simulink model "bms_unified"  (R2024b)
settings: Solver=FixedStepDiscrete  StartTime=0.0  StopTime=BMS_StopTime  FixedStep=1  RelTol=1e-3
InitFcn:
  | bms_setup('unified')
values from neighbouring files (symbols this model uses):
  BMS_Q : value not decoded    [bms_data.sldd]
  BMS_R = 0.001474701    [bms_data.sldd]
  NASA_Q : value not decoded    [bms_data.sldd]
  NASA_R = 0.009881778    [bms_data.sldd]
undefined symbols (not defined in the file or in its folder): BMS_FaultMode, BMS_InjectFaultsOnReplay, BMS_Seed, BMS_SOC0, BMS_SOC_Guess, BMS_Source, NASA_SOC_Guess
settings Model: DataDictionary=bms_data.sldd  Creator=sande  LastModifiedBy=sande
settings DataIOCC: SaveOutput=off
settings DebuggingCC: SignalInfNanChecking=error  AlgebraicLoopMsg=error  ArtificialAlgebraicLoopMsg=error  UnconnectedInputMsg=error  UnconnectedOutputMsg=error  UnconnectedLineMsg=error  BusObjectLabelMismatch=error  StrictBusMsg=ErrorOnBusTreatedAsVector
settings HardwareCC: ProdBitPerPointer=32  ProdBitPerSizeT=32  ProdBitPerPtrDiffT=32  ProdLargestAtomicInteger=Long  ProdLargestAtomicFloat=Double  ProdWordSize=32  ProdHWDeviceType=ARM Compatible->ARM Cortex

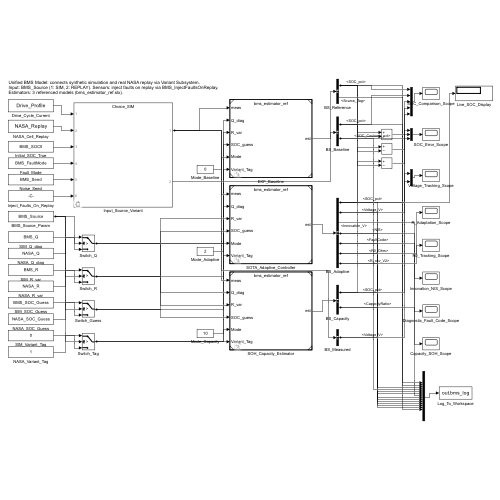
[thumbnail: Simulink's stored preview of the top-level diagram]
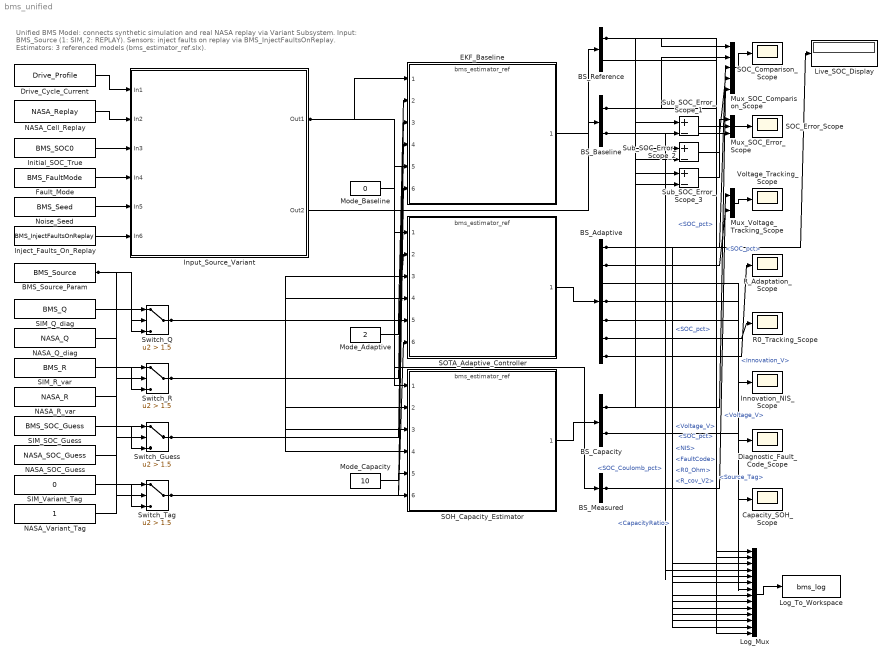
== system bms_unified ==
  note: Unified BMS Model: connects synthetic simulation and real NASA replay via Variant Subsystem.
      | Input: BMS_Source (1: SIM, 2: REPLAY). Sensors: inject faults on replay via BMS_InjectFaultsOnReplay.
      | Estimators: 3 referenced models (bms_estimator_ref.slx).
  BMS_Source_Param : Constant  Value=BMS_Source  SampleTime=-1
  BS_Adaptive : BusSelector  OutputSignals=SOC_pct,Voltage_V,Innovation_V,NIS,FaultCode,R0_Ohm,R_cov_V2
  BS_Baseline : BusSelector  OutputSignals=SOC_pct,SOC_Coulomb_pct
  BS_Capacity : BusSelector  OutputSignals=SOC_pct,CapacityRatio
  BS_Measured : BusSelector  OutputSignals=Voltage_V
  BS_Reference : BusSelector  OutputSignals=SOC_pct,Source_Tag
  Capacity_SOH_Scope : Scope
      settings: Description=Estimated capacity ratio (SOH)
  Diagnostic_Fault_Code_Scope : Scope
      settings: Description=Diagnostic bit-mask
  Drive_Cycle_Current : FromWorkspace  VariableName=Drive_Profile  SampleTime=1  Interpolate=off  OutputAfterFinalValue=Holding final value
  EKF_Baseline : ModelReference  ModelNameDialog=bms_estimator_ref  SimulationMode=Normal  ModelReferenceVersion=1.2
  Fault_Mode : Constant  Value=BMS_FaultMode  SampleTime=-1
  Initial_SOC_True : Constant  Value=BMS_SOC0  SampleTime=-1
  Inject_Faults_On_Replay : Constant  Value=BMS_InjectFaultsOnReplay  SampleTime=-1
  Innovation_NIS_Scope : Scope
      settings: Description=NIS (expect ~1)
  Input_Source_Variant : Subsystem  Variant=on
  Live_SOC_Display : Display
  Log_Mux : Mux  Inputs=14
  Log_To_Workspace : ToWorkspace  VariableName=bms_log  SampleTime=-1
  Mode_Adaptive : Constant  Value=2  SampleTime=-1
  Mode_Baseline : Constant  Value=0  SampleTime=-1
  Mode_Capacity : Constant  Value=10  SampleTime=-1
  Mux_SOC_Comparison_Scope : Mux  Inputs=5
  Mux_SOC_Error_Scope : Mux  Inputs=3
  Mux_Voltage_Tracking_Scope : Mux  Inputs=2
  NASA_Cell_Replay : FromWorkspace  VariableName=NASA_Replay  SampleTime=1  Interpolate=off  OutputAfterFinalValue=Holding final value
  NASA_Q_diag : Constant  Value=NASA_Q  SampleTime=-1
  NASA_R_var : Constant  Value=NASA_R  SampleTime=-1
  NASA_SOC_Guess : Constant  Value=NASA_SOC_Guess  SampleTime=-1
  NASA_Variant_Tag : Constant  SampleTime=-1
  Noise_Seed : Constant  Value=BMS_Seed  SampleTime=-1
  R0_Tracking_Scope : Scope
      settings: Description=R0 used by adaptive model [ohm]
  R_Adaptation_Scope : Scope
      settings: Description=Sage-Husa measurement-noise variance R
  SIM_Q_diag : Constant  Value=BMS_Q  SampleTime=-1
  SIM_R_var : Constant  Value=BMS_R  SampleTime=-1
  SIM_SOC_Guess : Constant  Value=BMS_SOC_Guess  SampleTime=-1
  SIM_Variant_Tag : Constant  Value=0  SampleTime=-1
  SOC_Comparison_Scope : Scope
      settings: Description=Reference SOC | EKF | Adaptive EKF | Coulomb Counting | EKF+capacity
  SOC_Error_Scope : Scope
      settings: Description=EKF error | Adaptive EKF error | EKF+capacity error [%]
  SOH_Capacity_Estimator : ModelReference  ModelNameDialog=bms_estimator_ref  SimulationMode=Normal  ModelReferenceVersion=1.2
  SOTA_Adaptive_Controller : ModelReference  ModelNameDialog=bms_estimator_ref  SimulationMode=Normal  ModelReferenceVersion=1.2
  Sub_SOC_Error_Scope_1 : Sum  Inputs=+-
  Sub_SOC_Error_Scope_2 : Sum  Inputs=+-
  Sub_SOC_Error_Scope_3 : Sum  Inputs=+-
  Switch_Guess : Switch  Criteria=u2 > Threshold  Threshold=1.5  SaturateOnIntegerOverflow=off  InputSameDT=off
  Switch_Q : Switch  Criteria=u2 > Threshold  Threshold=1.5  SaturateOnIntegerOverflow=off  InputSameDT=off
  Switch_R : Switch  Criteria=u2 > Threshold  Threshold=1.5  SaturateOnIntegerOverflow=off  InputSameDT=off
  Switch_Tag : Switch  Criteria=u2 > Threshold  Threshold=1.5  SaturateOnIntegerOverflow=off  InputSameDT=off
  Voltage_Tracking_Scope : Scope
      settings: Description=Measured V | Adaptive EKF predicted V
  wires:
  NASA_Q_diag/1 -> Switch_Q/1
  BMS_Source_Param/1 -> Switch_Q/2, Switch_R/2, Switch_Guess/2, Switch_Tag/2
  SIM_Q_diag/1 -> Switch_Q/3
  NASA_R_var/1 -> Switch_R/1
  SIM_R_var/1 -> Switch_R/3
  NASA_SOC_Guess/1 -> Switch_Guess/1
  SIM_SOC_Guess/1 -> Switch_Guess/3
  NASA_Variant_Tag/1 -> Switch_Tag/1
  SIM_Variant_Tag/1 -> Switch_Tag/3
  Drive_Cycle_Current/1 -> Input_Source_Variant/1(In1)
  NASA_Cell_Replay/1 -> Input_Source_Variant/2(In2)
  Initial_SOC_True/1 -> Input_Source_Variant/3(In3)
  Fault_Mode/1 -> Input_Source_Variant/4(In4)
  Noise_Seed/1 -> Input_Source_Variant/5(In5)
  Inject_Faults_On_Replay/1 -> Input_Source_Variant/6(In6)
  Input_Source_Variant/1(Out1) -> EKF_Baseline/1, SOTA_Adaptive_Controller/1, SOH_Capacity_Estimator/1, BS_Measured/1
  Switch_Q/1 -> EKF_Baseline/2, SOTA_Adaptive_Controller/2, SOH_Capacity_Estimator/2
  Switch_R/1 -> EKF_Baseline/3, SOTA_Adaptive_Controller/3, SOH_Capacity_Estimator/3
  Switch_Guess/1 -> EKF_Baseline/4, SOTA_Adaptive_Controller/4, SOH_Capacity_Estimator/4
  Switch_Tag/1 -> EKF_Baseline/6, SOTA_Adaptive_Controller/6, SOH_Capacity_Estimator/6
  Mode_Baseline/1 -> EKF_Baseline/5
  Mode_Adaptive/1 -> SOTA_Adaptive_Controller/5
  Mode_Capacity/1 -> SOH_Capacity_Estimator/5
  Input_Source_Variant/2(Out2) -> BS_Reference/1
  EKF_Baseline/1 -> BS_Baseline/1
  SOTA_Adaptive_Controller/1 -> BS_Adaptive/1
  SOH_Capacity_Estimator/1 -> BS_Capacity/1
  BS_Reference/1 -> Mux_SOC_Comparison_Scope/1, Sub_SOC_Error_Scope_1/2, Sub_SOC_Error_Scope_2/2, Sub_SOC_Error_Scope_3/2, Log_Mux/1  "<SOC_pct>"
  BS_Baseline/1 -> Mux_SOC_Comparison_Scope/2, Sub_SOC_Error_Scope_1/1, Log_Mux/2  "<SOC_pct>"
  BS_Adaptive/1 -> Mux_SOC_Comparison_Scope/3, Sub_SOC_Error_Scope_2/1, Live_SOC_Display/1, Log_Mux/3  "<SOC_pct>"
  BS_Baseline/2 -> Mux_SOC_Comparison_Scope/4, Log_Mux/4  "<SOC_Coulomb_pct>"
  BS_Capacity/1 -> Mux_SOC_Comparison_Scope/5, Sub_SOC_Error_Scope_3/1, Log_Mux/12  "<SOC_pct>"
  Mux_SOC_Comparison_Scope/1 -> SOC_Comparison_Scope/1
  Sub_SOC_Error_Scope_1/1 -> Mux_SOC_Error_Scope/1
  Sub_SOC_Error_Scope_2/1 -> Mux_SOC_Error_Scope/2
  Sub_SOC_Error_Scope_3/1 -> Mux_SOC_Error_Scope/3
  Mux_SOC_Error_Scope/1 -> SOC_Error_Scope/1
  BS_Measured/1 -> Mux_Voltage_Tracking_Scope/1, Log_Mux/5  "<Voltage_V>"
  BS_Adaptive/2 -> Mux_Voltage_Tracking_Scope/2, Log_Mux/6  "<Voltage_V>"
  Mux_Voltage_Tracking_Scope/1 -> Voltage_Tracking_Scope/1
  BS_Adaptive/7 -> R_Adaptation_Scope/1, Log_Mux/11  "<R_cov_V2>"
  BS_Adaptive/6 -> R0_Tracking_Scope/1, Log_Mux/10  "<R0_Ohm>"
  BS_Adaptive/4 -> Innovation_NIS_Scope/1, Log_Mux/8  "<NIS>"
  BS_Adaptive/5 -> Diagnostic_Fault_Code_Scope/1, Log_Mux/9  "<FaultCode>"
  BS_Capacity/2 -> Capacity_SOH_Scope/1, Log_Mux/13  "<CapacityRatio>"
  BS_Adaptive/3 -> Log_Mux/7  "<Innovation_V>"
  BS_Reference/2 -> Log_Mux/14  "<Source_Tag>"
  Log_Mux/1 -> Log_To_Workspace/1

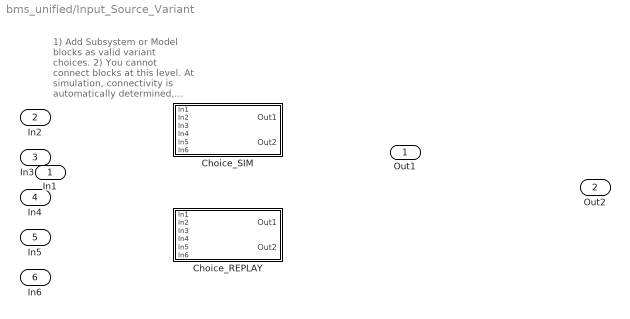
== system bms_unified/Input_Source_Variant ==
  note: 1) Add Subsystem or Model blocks as valid variant choices.
      | 2) You cannot connect blocks at this level. At simulation, connectivity is automatically
      | determined, based on the active variant and port name matching.
  In1 : Inport
  In2 : Inport  Port=2
  In3 : Inport  Port=3
  In4 : Inport  Port=4
  In5 : Inport  Port=5
  In6 : Inport  Port=6
  Choice_REPLAY : Subsystem  VariantControl=BMS_Source == 2
  Choice_SIM : Subsystem  VariantControl=BMS_Source == 1
  Out1 : Outport  OutDataTypeStr=Bus: BMS_Measurement
  Out2 : Outport  Port=2  OutDataTypeStr=Bus: BMS_Reference

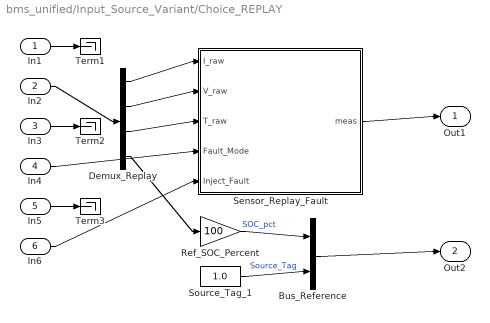
== system bms_unified/Input_Source_Variant/Choice_REPLAY ==
  In1 : Inport
  In2 : Inport  Port=2
  In3 : Inport  Port=3
  In4 : Inport  Port=4
  In5 : Inport  Port=5
  In6 : Inport  Port=6
  Bus_Reference : BusCreator  Inputs=2  OutDataTypeStr=Bus: BMS_Reference
  Demux_Replay : Demux
  Ref_SOC_Percent : Gain  Gain=100
  Sensor_Replay_Fault : MATLAB Function  TreatAsAtomicUnit=on
  Source_Tag_1 : Constant  Value=1.0
  Term1 : Terminator
  Term2 : Terminator
  Term3 : Terminator
  Out1 : Outport  OutDataTypeStr=Bus: BMS_Measurement
  Out2 : Outport  Port=2  OutDataTypeStr=Bus: BMS_Reference
  wires:
  In1/1 -> Term1/1
  In3/1 -> Term2/1
  In5/1 -> Term3/1
  In2/1 -> Demux_Replay/1
  Demux_Replay/1 -> Sensor_Replay_Fault/1(I_raw)
  Demux_Replay/2 -> Sensor_Replay_Fault/2(V_raw)
  Demux_Replay/3 -> Sensor_Replay_Fault/3(T_raw)
  In4/1 -> Sensor_Replay_Fault/4(Fault_Mode)
  In6/1 -> Sensor_Replay_Fault/5(Inject_Fault)
  Sensor_Replay_Fault/1(meas) -> Out1/1
  Demux_Replay/4 -> Ref_SOC_Percent/1
  Ref_SOC_Percent/1 -> Bus_Reference/1  "SOC_pct"
  Source_Tag_1/1 -> Bus_Reference/2  "Source_Tag"
  Bus_Reference/1 -> Out2/1

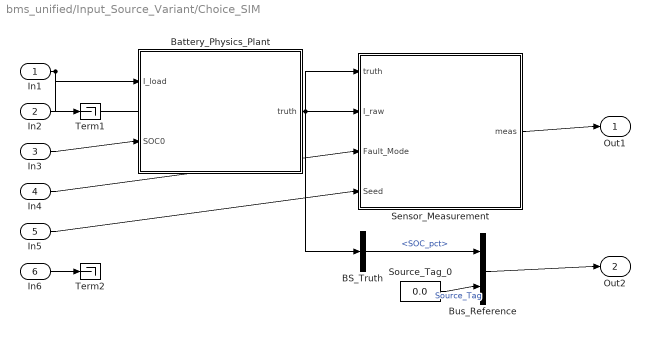
== system bms_unified/Input_Source_Variant/Choice_SIM ==
  In1 : Inport
  In2 : Inport  Port=2
  In3 : Inport  Port=3
  In4 : Inport  Port=4
  In5 : Inport  Port=5
  In6 : Inport  Port=6
  BS_Truth : BusSelector  OutputSignals=SOC_pct
  Battery_Physics_Plant : MATLAB Function  TreatAsAtomicUnit=on
  Bus_Reference : BusCreator  Inputs=2  OutDataTypeStr=Bus: BMS_Reference
  Sensor_Measurement : MATLAB Function  TreatAsAtomicUnit=on
  Source_Tag_0 : Constant  Value=0.0
  Term1 : Terminator
  Term2 : Terminator
  Out1 : Outport  OutDataTypeStr=Bus: BMS_Measurement
  Out2 : Outport  Port=2  OutDataTypeStr=Bus: BMS_Reference
  wires:
  In2/1 -> Term1/1
  In6/1 -> Term2/1
  In1/1 -> Battery_Physics_Plant/1(I_load), Sensor_Measurement/2(I_raw)
  In3/1 -> Battery_Physics_Plant/2(SOC0)
  Battery_Physics_Plant/1(truth) -> Sensor_Measurement/1(truth), BS_Truth/1
  In4/1 -> Sensor_Measurement/3(Fault_Mode)
  In5/1 -> Sensor_Measurement/4(Seed)
  Sensor_Measurement/1(meas) -> Out1/1
  BS_Truth/1 -> Bus_Reference/1  "<SOC_pct>"
  Source_Tag_0/1 -> Bus_Reference/2  "Source_Tag"
  Bus_Reference/1 -> Out2/1

== matlab function bms_unified/Input_Source_Variant/Choice_SIM/Sensor_Measurement ==
  data: truth input Bus: BMS_PlantTruth; meas output Bus: BMS_Measurement; I_raw input; Fault_Mode input; Seed input
function meas = Sensor_Measurement(truth, I_raw, Fault_Mode, Seed)
%#codegen
% Noisy 12-bit-class sensors with injectable faults. Algorithm: lib/bms_sensor_step.m (seeded, reproducible)
% Input: bus BMS_PlantTruth. Output: bus BMS_Measurement
P = coder.const(bms_params('synthetic'));
persistent ss k;
if isempty(ss)
    ss = bms_seed(Seed);  k = 0.0;
end
k = k + 1.0;
[Vm, Im, Tm, ss] = bms_sensor_step(truth.Voltage_V, I_raw, truth.Temperature_K, k, ss, P, Fault_Mode);
meas.Voltage_V = Vm;
meas.Current_A = Im;
meas.Temperature_K = Tm;

== matlab function bms_unified/Input_Source_Variant/Choice_SIM/Battery_Physics_Plant ==
  data: I_load input; truth output Bus: BMS_PlantTruth; SOC0 input
function truth = Battery_Physics_Plant(I_load, SOC0)
%#codegen
% 2-RC Arrhenius cell with capacity/resistance mismatch (see bms_params). Algorithm: lib/bms_plant_step.m
% Output: bus BMS_PlantTruth
P = coder.const(bms_params('synthetic'));
persistent x k;
if isempty(x)
    x = [SOC0; 0.0; 0.0];  k = 0.0;
end
k = k + 1.0;
T = bms_temp_profile(k);
[x, Vt] = bms_plant_step(x, I_load, T, P);
truth.SOC_pct = 100.0 * x(1);
truth.Voltage_V = Vt;
truth.Temperature_K = T;

== matlab function bms_unified/Input_Source_Variant/Choice_REPLAY/Sensor_Replay_Fault ==
  data: I_raw input; meas output Bus: BMS_Measurement; V_raw input; T_raw input; Fault_Mode input; Inject_Fault input
function meas = Sensor_Replay_Fault(I_raw, V_raw, T_raw, Fault_Mode, Inject_Fault)
%#codegen
% Common sensor interface for REPLAY: passes real NASA signals cleanly unless
% BMS_InjectFaultsOnReplay is active.
P = coder.const(bms_params('nasa'));
persistent k;
if isempty(k),  k = 0.0;  end
k = k + 1.0;
Vm = V_raw;  Im = I_raw;  Tm = T_raw;
if Inject_Fault > 0.5 && k >= P.fault_k0 && k <= P.fault_k1
    if Fault_Mode == 1.0
        Im = Im + P.fault_I_offset;
    elseif Fault_Mode == 2.0
        if mod(k, 25.0) == 0.0
            Vm = Vm + P.fault_V_spike * (1.0 - 2.0 * mod(k / 25.0, 2.0));
        end
    elseif Fault_Mode == 3.0
        Tm = P.fault_T_stuck;
    end
end
meas.Voltage_V = Vm;
meas.Current_A = Im;
meas.Temperature_K = Tm;
